simulink model "BP_RBFNN"  (R2022a)
settings: Solver=FixedStepAuto  StartTime=0.0  StopTime=100  FixedStep=0.001  RelTol=1e-3
settings Model: Creator=Userx  LastModifiedBy=Userx

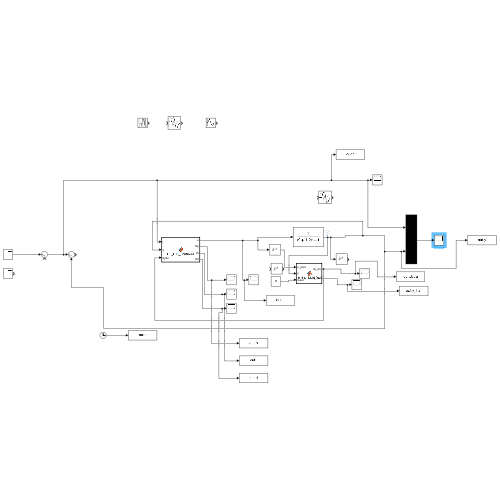
[thumbnail: Simulink's stored preview of the top-level diagram]
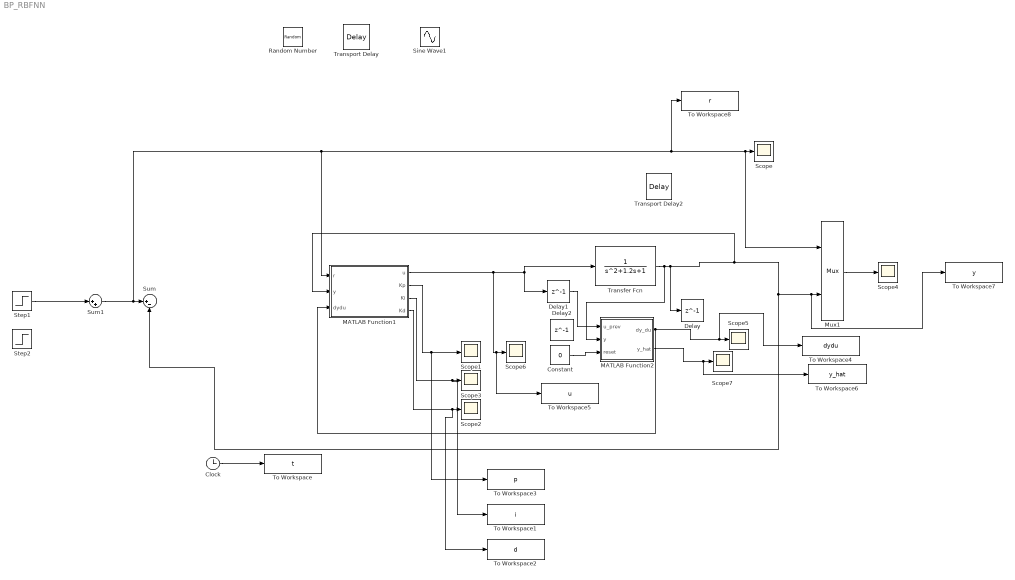
== system BP_RBFNN ==
  Clock : Clock
  Constant : Constant  Value=0
  Delay : Delay  DelayLength=1
  Delay1 : Delay  DelayLength=1
  Delay2 : Delay  DelayLength=1
  MATLAB Function1 : MATLAB Function  TreatAsAtomicUnit=on
  MATLAB Function2 : MATLAB Function  TreatAsAtomicUnit=on
  Mux1 : Mux  Inputs=2
  Random Number : RandomNumber  Variance=0.01  SampleTime=0.1
  Scope{,1..7} (8 alike) : Scope
  Sine Wave1 : Sin  Frequency=0.10  SampleTime=0
  Step1 : Step  Time=0  SampleTime=0
  Step2 : Step  Time=10  SampleTime=0
  Sum : Sum  Inputs=|+-
  Sum1 : Sum  Inputs=|++
  To Workspace : ToWorkspace  VariableName=t  SampleTime=-1
  To Workspace1 : ToWorkspace  VariableName=i  SampleTime=-1
  To Workspace2 : ToWorkspace  VariableName=d  SampleTime=-1
  To Workspace3 : ToWorkspace  VariableName=p  SampleTime=-1
  To Workspace4 : ToWorkspace  VariableName=dydu  SampleTime=-1
  To Workspace5 : ToWorkspace  VariableName=u  SampleTime=-1
  To Workspace6 : ToWorkspace  VariableName=y_hat  SampleTime=-1
  To Workspace7 : ToWorkspace  VariableName=y  SampleTime=-1
  To Workspace8 : ToWorkspace  VariableName=r  SampleTime=-1
  Transfer Fcn : TransferFcn  Denominator=[1 1.2 1]
  Transport Delay : TransportDelay
  Transport Delay2 : TransportDelay  DelayTime=0.1
  wires:
  Mux1/1 -> Scope4/1
  Clock/1 -> To Workspace/1
  Step1/1 -> Sum1/1
  Sum1/1 -> MATLAB Function1/1(r), To Workspace8/1, Mux1/1, Scope/1, Sum/1
  MATLAB Function2/1(dy_du) -> MATLAB Function1/3(dydu), To Workspace4/1, Scope5/1
  MATLAB Function1/2(Kp) -> Scope1/1, To Workspace3/1
  MATLAB Function1/3(Ki) -> To Workspace1/1, Scope3/1
  MATLAB Function1/4(Kd) -> To Workspace2/1, Scope2/1
  MATLAB Function1/1(u) -> Transfer Fcn/1, Delay1/1, To Workspace5/1, Scope6/1
  Transfer Fcn/1 -> MATLAB Function2/2(y), MATLAB Function1/2(y), Sum/2, To Workspace7/1, Mux1/2, Delay/1
  Constant/1 -> MATLAB Function2/3(reset)
  MATLAB Function2/2(y_hat) -> To Workspace6/1, Scope7/1
  Delay1/1 -> MATLAB Function2/1(u_prev)

== matlab function BP_RBFNN/MATLAB Function1 ==
  settings: updateMethod=DISCRETE
  data: r input; u output; y input; Kp output; Ki output; Kd output; dydu input
function [u, Kp, Ki, Kd] = BP_PID_Controller(r, y, dydu)
% =========================================================================
% BP神经网络PID参数自整定控制器 (Simulink MATLAB Function Block)
% Jacobian ∂y/∂u 由外部 RBF 辨识器提供
% =========================================================================
%
% 网络结构：
%   输入层  (3个神经元)：误差 e(k)、误差变化率 de(k)、误差积分 ei(k)
%   隐含层  (5个神经元)：激活函数 Leaky ReLU
%   输出层  (3个神经元)：激活函数 sigmoid，对应 Kp、Ki、Kd
%
% 端口说明：
%   输入端口：
%     r    - 参考指令（设定值）
%     y    - 被控对象输出（测量值/反馈量）
%     dydu - RBF辨识器提供的雅可比 ∂y/∂u（标量）
%
%   输出端口：
%     u  - PID控制量（输出给执行器/被控对象）
%     Kp - 比例系数（实时监控）
%     Ki - 积分系数（实时监控）
%     Kd - 微分系数（实时监控）
%
% =========================================================================

%% ---------- 持久变量声明（网络权值 & 状态量）----------
persistent w_ih dw_ih   % 输入层→隐含层 权值矩阵 & 上次增量（动量项）
persistent w_ho dw_ho   % 隐含层→输出层 权值矩阵 & 上次增量（动量项）
persistent e_1 e_2      % e(k-1), e(k-2)：计算增量式PID所需历史误差
persistent u_1          % u(k-1)：上一时刻控制量
persistent Oh           % 隐含层输出（供反向传播复用）
persistent Oo           % 输出层输出（供反向传播复用）
persistent ei_acc       % 误差积分累加器（真积分）
persistent step_count     % 步数计数器，学习率衰减用
persistent u_smooth       % 控制量指数平滑值

%% ---------- 超参数 ----------
n_in  = 3;   % 输入层神经元数
n_h   = 5;   % 隐含层神经元数
n_out = 3;   % 输出层神经元数（固定为3，对应 Kp/Ki/Kd）

lr0      = 0.01;    % 初始学习率
lr_decay = 0.0005;  % 指数衰减速率: lr = lr0 * exp(-step*ts*lr_decay)
alpha = 0.05;   % 动量系数 α
smooth_factor = 0.3;  % 控制量指数平滑因子 (0~1，越小越平滑)

ts = 0.01;   % 采样周期（与 Simulink 步长一致）

% PID 参数取值范围
Kp_min = 0.0;  Kp_max = 15.0;
Ki_min = 0.0;  Ki_max =  5.0;
Kd_min = 0.0;  Kd_max =  5.0;

% 控制量限幅
u_max =  10.0;
u_min = -10.0;

%% ---------- 首次调用：初始化权值和状态 ----------
if isempty(w_ih)
    rng(1);
    % Xavier 初始化：N(0, sqrt(2/(fan_in+fan_out)))
    w_ih  = sqrt(2/(n_in + n_h)) * randn(n_h, n_in + 1);
    dw_ih = zeros(n_h,  n_in + 1);
    w_ho  = sqrt(2/(n_h + n_out)) * randn(n_out, n_h + 1);
    dw_ho = zeros(n_out, n_h  + 1);
    e_1 = 0;   e_2 = 0;
    u_1 = 0;
    Oh     = zeros(n_h,   1);
    Oo     = 0.5 * ones(n_out, 1);
    ei_acc = 0;
    step_count = 0;
    u_smooth = 0;
end

% 学习率指数衰减
lr = lr0 * exp(-step_count * ts * lr_decay);

%% ---------- Step 1：计算当前误差 ----------
e  = r - y;                    % 跟踪误差 e(k)
de = e - e_1;                  % 误差变化量

% 真积分累加 + 抗饱和
if ~((u_1 >= u_max && e > 0) || (u_1 <= u_min && e < 0))
    ei_acc = ei_acc + e * ts;
end
ei_acc = max(-3.0, min(3.0, ei_acc));
ei = ei_acc;

Xi = [e; de; ei];              % 3×1

%% ---------- Step 2：前向传播 ----------
% 隐含层（Leaky ReLU 激活，负斜率 0.01）
net_h = w_ih * [Xi; 1];       % [n_h × 1]，+1 为偏置输入
Oh    = max(0.01*net_h, net_h);  % [n_h × 1]

% 输出层（sigmoid 激活，输出范围 (0, 1)）
net_o = w_ho * [Oh; 1];       % [n_out × 1]
Oo    = 1 ./ (1 + exp(-net_o)); % [n_out × 1]

%% ---------- Step 3：映射到 PID 参数 ----------
Kp = Kp_min + (Kp_max - Kp_min) * Oo(1);
Ki = Ki_min + (Ki_max - Ki_min) * Oo(2);
Kd = Kd_min + (Kd_max - Kd_min) * Oo(3);

%% ---------- Step 4：增量式PID控制律 ----------
delta_u = Kp * de + Ki * e + Kd * (e - 2*e_1 + e_2);

u = u_1 + delta_u;

% 控制量限幅
u = max(u_min, min(u_max, u));

% 输出指数平滑（抑制高频振荡）
u_smooth = smooth_factor * u + (1 - smooth_factor) * u_smooth;
u = u_smooth;

%% ---------- Step 5：反向传播在线更新权值 ----------
%
% 代价函数：J = 0.5 * e(k)^2
% Jacobian ∂J/∂u = -e * dydu   ← dydu 由外部 RBF 辨识器提供
dJ_du = -e * dydu;

% 各 K 对控制量的偏导（增量式 PID）
dU_dKp = de;
dU_dKi = e;
dU_dKd = e - 2*e_1 + e_2;
dU_dK  = [dU_dKp; dU_dKi; dU_dKd];   % [3 × 1]

% Kp/Ki/Kd 对 Oo 的偏导（线性映射）
dK_dOo = [Kp_max - Kp_min;
           Ki_max - Ki_min;
           Kd_max - Kd_min];            % [3 × 1]

% sigmoid 导数：dOo/dnet_o = Oo*(1-Oo)
d_sigmoid = Oo .* (1 - Oo);            % [3 × 1]

% 输出层误差信号 δ_o（[3 × 1]）
delta_o = dJ_du * dU_dK .* dK_dOo .* d_sigmoid;

% 输出层权值更新（含动量项）
grad_w_ho  = delta_o * [Oh; 1]';       % [3 × (n_h+1)]
new_dw_ho  = -lr * grad_w_ho + alpha * dw_ho;
w_ho       = w_ho + new_dw_ho;
dw_ho      = new_dw_ho;

% 隐含层误差信号 δ_h（[n_h × 1]）
d_leaky = ones(n_h, 1); d_leaky(net_h <= 0) = 0.01;  % LeakyReLU 导数
delta_h    = (w_ho(:, 1:n_h)' * delta_o) .* d_leaky;  % [n_h × 1]

% 梯度裁剪
delta_o = max(-1.0, min(1.0, delta_o));
delta_h = max(-1.0, min(1.0, delta_h));

% 输入层→隐含层权值更新（含动量项）
grad_w_ih  = delta_h * [Xi; 1]';      % [n_h × (n_in+1)]
new_dw_ih  = -lr * grad_w_ih + alpha * dw_ih;
w_ih       = w_ih + new_dw_ih;
dw_ih      = new_dw_ih;

%% ---------- Step 6：状态更新 ----------
e_2 = e_1;
e_1 = e;
u_1 = u;
step_count = step_count + 1;

end   % function BP_PID_Controller

== matlab function BP_RBFNN/MATLAB Function2 ==
  settings: updateMethod=DISCRETE
  data: u_prev input; y input; reset input; dy_du output; y_hat output
function [dy_du, y_hat] = rbf_online_identification(u_prev, y, reset)
% RBF神经网络在线辨识 — 为 BP-PID 提供 ∂y/∂u
%
% 输入:
%   u_prev — u(k-1)，控制量经 Unit Delay 后接入
%   y      — y(k)，被控对象当前输出
%   reset  — 复位信号，接常数 0
%
% 输出:
%   dy_du  — 雅可比 ∂y/∂u
%   y_hat  — RBF 预测输出

persistent W C Sigma dW_prev dC_prev dSig_prev y1 y2 u2 gain init_flag

%% ===== 超参数 =====
M       = 10;     % RBF 隐层节点数（从 8 增至 10）
n       = 4;      % 输入维度 [y(k-1), y(k-2), u(k-1), u(k-2)]
eta_w   = 0.10;   % W 学习率（从 0.30 降至 0.10）
eta_c   = 0.08;   % C 学习率（从 0.05 提至 0.08）
eta_s   = 0.05;   % σ 学习率
mu_w    = 0.05;   % W 动量系数
mu_c    = 0.02;   % C 动量系数
mu_s    = 0.02;   % σ 动量系数
sig_min = 0.02;   % σ 下限

%% ===== 初始化 =====
if isempty(init_flag) || reset > 0.5
    % 输入归一化增益：将各维映射到约 [-1, 1]
    % y 范围 ~ [0, 2] → gain=1.0（以 0 为中心约 ±1）
    % u 范围 ~ [-10, 10] → gain=0.1（映射到 ±1）
    gain = [0.8; 0.8; 0.1; 0.1];

    W     = 0.1 * randn(1, M);
    % 中心在归一化空间初始化为 [-1, 1] 均匀分布
    rng(0);
    C     = 2*(rand(M, n)-0.5);   % [-1, 1]
    Sigma = 1.5 * ones(M, 1);
    dW_prev   = zeros(1, M);
    dC_prev   = zeros(M, n);
    dSig_prev = zeros(M, 1);
    y1 = 0; y2 = 0; u2 = 0;
    init_flag = true;
end

%% ===== 构造归一化输入 =====
x_raw = [y1; y2; double(u_prev); u2];  % 4×1
x = x_raw .* gain;                      % 归一化

%% ===== 前向传播 =====
D     = bsxfun(@minus, x', C);              % M×n
dist2 = sum(D .^ 2, 2);                     % M×1
H     = exp(-dist2 ./ (2 * Sigma .^ 2));    % M×1
y_hat = W * H;                              % 标量

%% ===== 辨识误差 =====
e = double(y) - y_hat;

%% ===== 梯度计算 =====
grad_W = -e * H';
scale  = (W .* H') ./ (Sigma .^ 2)';
grad_C = -e * bsxfun(@times, D, scale');
grad_S = -e * (W' .* H .* dist2 ./ (Sigma .^ 3));

%% ===== 带动量的参数更新 =====
dW = -eta_w * grad_W + mu_w * dW_prev;
dC = -eta_c * grad_C + mu_c * dC_prev;
dS = -eta_s * grad_S + mu_s * dSig_prev;

W     = W + dW;
C     = C + dC;
Sigma = max(Sigma + dS, sig_min);

dW_prev   = dW;
dC_prev   = dC;
dSig_prev = dS;

%% ===== 雅可比 ∂ŷ/∂u(k-1) =====
% 归一化空间的偏导 * gain(3) 还原到原始空间
dy_du_norm = sum(W' .* H .* (-D(:,3) ./ Sigma .^ 2));
dy_du = dy_du_norm * gain(3);

% 下限保护
if abs(dy_du) < 1e-4
    dy_du = sign(dy_du + eps) * 1e-4;
end

%% ===== 更新延迟寄存器 =====
y2 = y1;
y1 = double(y);
u2 = double(u_prev);

end
